simulink model "Kirov_physics"  (R2024b)
settings: Solver=FixedStepDiscrete  StartTime=0.0  StopTime=inf  FixedStep=dt  RelTol=1e-3
undefined symbols (not defined in the file): accel_O, airspeed_bp, alpha_B, alpha_bp, alphaFull, alphaOff, b, battery_capacity_bp, battery_current_bp, battery_initial_capacity_mAh, battery_voltage_table, beta_bp, betaFull, betaOff, brake, brakes, c, channels, CLa, Clb, Clp, CLq, Clr, Cma, Cmq, Cnb, Cnp, Cnr, current_table, DiscIntNeverNeededParam, dt, ELEV_bp, elevator, f, flap, flaps, FLAPS_bp, gear, heightFadeStart, heightOff, hgt_0, Inertia_body, Inertia_load, kInduced, L_aileron, L_throttle, LAILE_bp, lat_0, lon_0, M_aile, M_body, M_elev, M_flap, M_front_gear, M_load, M_main_gear, M_prop, M_rudd, M_spoiler, minWingHeight ... (+36)
libraries: sm_lib x673, simulink x58, nesl_utility x51, simulink_extras x24, uavmavlinklib x12, instrumentlib x4, vrlib x3, aerolibfltsims x3, sharedtransform x3, eeGeneralControl x2, aerolibutil x2, AP_Connector x2
(part 5 of 6)

== system Kirov_physics/Dynamics/Subsystem2 ==
  surface_input(deg) : Inport
  Degrees to Radians : simulink_extras/Transformations/Degrees to Radians
  Discrete Derivative : simulink/Quick Insert/Discrete/Discrete Derivative  gainval=1.0  ICPrevScaledInput=0.0  OutMin=[]  OutMax=[]  OutDataType=fixdt(1, 16)  OutScaling=2^-10  DoSatur=off
  Discrete Derivative1 : simulink/Quick Insert/Discrete/Discrete Derivative  gainval=1.0  ICPrevScaledInput=0.0  OutMin=[]  OutMax=[]  OutDataType=fixdt(1, 16)  OutScaling=2^-10  DoSatur=off
  Simulink-PS Converter : nesl_utility/Simulink-PS Converter  PhysicalDomain=network_engine_domain  SubClassName=ps_input  LeftPortType=input  RightPortType=output  PseudoPeriodic=off  Frequencies=[]  NoiseDistribution=none  NoiseParameters=[]  Unit=rad  AffineConversion=off  FilteringAndDerivatives=provide  SimscapeFilterOrder=1  InputFilterTimeConstant=0.001  UdotUserProvided=2
  surface_output : PMIOPort  Side=Right
  wires:
  Degrees to Radians/1 -> Simulink-PS Converter/1, Discrete Derivative/1
  Discrete Derivative1/1 -> Simulink-PS Converter/3
  Discrete Derivative/1 -> Simulink-PS Converter/2, Discrete Derivative1/1
  surface_input(deg)/1 -> Degrees to Radians/1
  connections:
  Simulink-PS Converter/RConn1 -- surface_output/RConn1

== system Kirov_physics/Dynamics/Subsystem20 ==
  prop_rad : Inport
  Discrete Derivative : simulink/Quick Insert/Discrete/Discrete Derivative  gainval=1.0  ICPrevScaledInput=0.0  OutMin=[]  OutMax=[]  OutDataType=fixdt(1, 16)  OutScaling=2^-10  DoSatur=off
  Discrete Derivative1 : simulink/Quick Insert/Discrete/Discrete Derivative  gainval=1.0  ICPrevScaledInput=0.0  OutMin=[]  OutMax=[]  OutDataType=fixdt(1, 16)  OutScaling=2^-10  DoSatur=off
  Simulink-PS Converter : nesl_utility/Simulink-PS Converter  PhysicalDomain=network_engine_domain  SubClassName=ps_input  LeftPortType=input  RightPortType=output  PseudoPeriodic=off  Frequencies=[]  NoiseDistribution=none  NoiseParameters=[]  Unit=rad  AffineConversion=off  FilteringAndDerivatives=provide  SimscapeFilterOrder=1  InputFilterTimeConstant=0.001  UdotUserProvided=2
  prop_output : PMIOPort  Side=Right
  wires:
  Discrete Derivative/1 -> Discrete Derivative1/1, Simulink-PS Converter/2
  Discrete Derivative1/1 -> Simulink-PS Converter/3
  prop_rad/1 -> Discrete Derivative/1, Simulink-PS Converter/1
  connections:
  Simulink-PS Converter/RConn1 -- prop_output/RConn1

== system Kirov_physics/Dynamics/Subsystem3 ==
  surface_input(deg) : Inport
  Degrees to Radians : simulink_extras/Transformations/Degrees to Radians
  Discrete Derivative : simulink/Quick Insert/Discrete/Discrete Derivative  gainval=1.0  ICPrevScaledInput=0.0  OutMin=[]  OutMax=[]  OutDataType=fixdt(1, 16)  OutScaling=2^-10  DoSatur=off
  Discrete Derivative1 : simulink/Quick Insert/Discrete/Discrete Derivative  gainval=1.0  ICPrevScaledInput=0.0  OutMin=[]  OutMax=[]  OutDataType=fixdt(1, 16)  OutScaling=2^-10  DoSatur=off
  Simulink-PS Converter : nesl_utility/Simulink-PS Converter  PhysicalDomain=network_engine_domain  SubClassName=ps_input  LeftPortType=input  RightPortType=output  PseudoPeriodic=off  Frequencies=[]  NoiseDistribution=none  NoiseParameters=[]  Unit=rad  AffineConversion=off  FilteringAndDerivatives=provide  SimscapeFilterOrder=1  InputFilterTimeConstant=0.001  UdotUserProvided=2
  surface_output : PMIOPort  Side=Right
  wires:
  Degrees to Radians/1 -> Simulink-PS Converter/1, Discrete Derivative/1
  Discrete Derivative1/1 -> Simulink-PS Converter/3
  Discrete Derivative/1 -> Simulink-PS Converter/2, Discrete Derivative1/1
  surface_input(deg)/1 -> Degrees to Radians/1
  connections:
  Simulink-PS Converter/RConn1 -- surface_output/RConn1

== system Kirov_physics/Dynamics/Subsystem4 ==
  surface_input(deg) : Inport
  Degrees to Radians : simulink_extras/Transformations/Degrees to Radians
  Discrete Derivative : simulink/Quick Insert/Discrete/Discrete Derivative  gainval=1.0  ICPrevScaledInput=0.0  OutMin=[]  OutMax=[]  OutDataType=fixdt(1, 16)  OutScaling=2^-10  DoSatur=off
  Discrete Derivative1 : simulink/Quick Insert/Discrete/Discrete Derivative  gainval=1.0  ICPrevScaledInput=0.0  OutMin=[]  OutMax=[]  OutDataType=fixdt(1, 16)  OutScaling=2^-10  DoSatur=off
  Simulink-PS Converter : nesl_utility/Simulink-PS Converter  PhysicalDomain=network_engine_domain  SubClassName=ps_input  LeftPortType=input  RightPortType=output  PseudoPeriodic=off  Frequencies=[]  NoiseDistribution=none  NoiseParameters=[]  Unit=rad  AffineConversion=off  FilteringAndDerivatives=provide  SimscapeFilterOrder=1  InputFilterTimeConstant=0.001  UdotUserProvided=2
  surface_output : PMIOPort  Side=Right
  wires:
  surface_input(deg)/1 -> Degrees to Radians/1
  Discrete Derivative/1 -> Discrete Derivative1/1, Simulink-PS Converter/2
  Discrete Derivative1/1 -> Simulink-PS Converter/3
  Degrees to Radians/1 -> Discrete Derivative/1, Simulink-PS Converter/1
  connections:
  Simulink-PS Converter/RConn1 -- surface_output/RConn1

== system Kirov_physics/Dynamics/Subsystem5 ==
  surface_input(deg) : Inport
  Degrees to Radians : simulink_extras/Transformations/Degrees to Radians
  Discrete Derivative : simulink/Quick Insert/Discrete/Discrete Derivative  gainval=1.0  ICPrevScaledInput=0.0  OutMin=[]  OutMax=[]  OutDataType=fixdt(1, 16)  OutScaling=2^-10  DoSatur=off
  Discrete Derivative1 : simulink/Quick Insert/Discrete/Discrete Derivative  gainval=1.0  ICPrevScaledInput=0.0  OutMin=[]  OutMax=[]  OutDataType=fixdt(1, 16)  OutScaling=2^-10  DoSatur=off
  Simulink-PS Converter : nesl_utility/Simulink-PS Converter  PhysicalDomain=network_engine_domain  SubClassName=ps_input  LeftPortType=input  RightPortType=output  PseudoPeriodic=off  Frequencies=[]  NoiseDistribution=none  NoiseParameters=[]  Unit=rad  AffineConversion=off  FilteringAndDerivatives=provide  SimscapeFilterOrder=1  InputFilterTimeConstant=0.001  UdotUserProvided=2
  surface_output : PMIOPort  Side=Right
  wires:
  surface_input(deg)/1 -> Degrees to Radians/1
  Discrete Derivative/1 -> Discrete Derivative1/1, Simulink-PS Converter/2
  Discrete Derivative1/1 -> Simulink-PS Converter/3
  Degrees to Radians/1 -> Discrete Derivative/1, Simulink-PS Converter/1
  connections:
  Simulink-PS Converter/RConn1 -- surface_output/RConn1

== system Kirov_physics/Dynamics/Subsystem6 ==
  surface_input(deg) : Inport
  Degrees to Radians : simulink_extras/Transformations/Degrees to Radians
  Discrete Derivative : simulink/Quick Insert/Discrete/Discrete Derivative  gainval=1.0  ICPrevScaledInput=0.0  OutMin=[]  OutMax=[]  OutDataType=fixdt(1, 16)  OutScaling=2^-10  DoSatur=off
  Discrete Derivative1 : simulink/Quick Insert/Discrete/Discrete Derivative  gainval=1.0  ICPrevScaledInput=0.0  OutMin=[]  OutMax=[]  OutDataType=fixdt(1, 16)  OutScaling=2^-10  DoSatur=off
  Simulink-PS Converter : nesl_utility/Simulink-PS Converter  PhysicalDomain=network_engine_domain  SubClassName=ps_input  LeftPortType=input  RightPortType=output  PseudoPeriodic=off  Frequencies=[]  NoiseDistribution=none  NoiseParameters=[]  Unit=rad  AffineConversion=off  FilteringAndDerivatives=provide  SimscapeFilterOrder=1  InputFilterTimeConstant=0.001  UdotUserProvided=2
  surface_output : PMIOPort  Side=Right
  wires:
  Degrees to Radians/1 -> Simulink-PS Converter/1, Discrete Derivative/1
  Discrete Derivative1/1 -> Simulink-PS Converter/3
  Discrete Derivative/1 -> Simulink-PS Converter/2, Discrete Derivative1/1
  surface_input(deg)/1 -> Degrees to Radians/1
  connections:
  Simulink-PS Converter/RConn1 -- surface_output/RConn1

== system Kirov_physics/Dynamics/Subsystem7 ==
  force_input(N) : Inport
  Discrete Derivative : simulink/Quick Insert/Discrete/Discrete Derivative  gainval=1.0  ICPrevScaledInput=0.0  OutMin=[]  OutMax=[]  OutDataType=fixdt(1, 16)  OutScaling=2^-10  DoSatur=off
  Discrete Derivative1 : simulink/Quick Insert/Discrete/Discrete Derivative  gainval=1.0  ICPrevScaledInput=0.0  OutMin=[]  OutMax=[]  OutDataType=fixdt(1, 16)  OutScaling=2^-10  DoSatur=off
  Simulink-PS Converter : nesl_utility/Simulink-PS Converter  PhysicalDomain=network_engine_domain  SubClassName=ps_input  LeftPortType=input  RightPortType=output  PseudoPeriodic=off  Frequencies=[]  NoiseDistribution=none  NoiseParameters=[]  Unit=N  AffineConversion=off  FilteringAndDerivatives=provide  SimscapeFilterOrder=1  InputFilterTimeConstant=0.001  UdotUserProvided=2
  force_output : PMIOPort  Side=Right
  wires:
  force_input(N)/1 -> Discrete Derivative/1, Simulink-PS Converter/1
  Discrete Derivative/1 -> Discrete Derivative1/1, Simulink-PS Converter/2
  Discrete Derivative1/1 -> Simulink-PS Converter/3
  connections:
  Simulink-PS Converter/RConn1 -- force_output/RConn1

== system Kirov_physics/Dynamics/Subsystem8 ==
  force_input(N) : Inport
  Discrete Derivative : simulink/Quick Insert/Discrete/Discrete Derivative  gainval=1.0  ICPrevScaledInput=0.0  OutMin=[]  OutMax=[]  OutDataType=fixdt(1, 16)  OutScaling=2^-10  DoSatur=off
  Discrete Derivative1 : simulink/Quick Insert/Discrete/Discrete Derivative  gainval=1.0  ICPrevScaledInput=0.0  OutMin=[]  OutMax=[]  OutDataType=fixdt(1, 16)  OutScaling=2^-10  DoSatur=off
  Simulink-PS Converter : nesl_utility/Simulink-PS Converter  PhysicalDomain=network_engine_domain  SubClassName=ps_input  LeftPortType=input  RightPortType=output  PseudoPeriodic=off  Frequencies=[]  NoiseDistribution=none  NoiseParameters=[]  Unit=N  AffineConversion=off  FilteringAndDerivatives=provide  SimscapeFilterOrder=1  InputFilterTimeConstant=0.001  UdotUserProvided=2
  force_output : PMIOPort  Side=Right
  wires:
  Discrete Derivative1/1 -> Simulink-PS Converter/3
  Discrete Derivative/1 -> Simulink-PS Converter/2, Discrete Derivative1/1
  force_input(N)/1 -> Simulink-PS Converter/1, Discrete Derivative/1
  connections:
  Simulink-PS Converter/RConn1 -- force_output/RConn1

== system Kirov_physics/Dynamics/Subsystem9 ==
  force_input(N) : Inport
  Discrete Derivative : simulink/Quick Insert/Discrete/Discrete Derivative  gainval=1.0  ICPrevScaledInput=0.0  OutMin=[]  OutMax=[]  OutDataType=fixdt(1, 16)  OutScaling=2^-10  DoSatur=off
  Discrete Derivative1 : simulink/Quick Insert/Discrete/Discrete Derivative  gainval=1.0  ICPrevScaledInput=0.0  OutMin=[]  OutMax=[]  OutDataType=fixdt(1, 16)  OutScaling=2^-10  DoSatur=off
  Simulink-PS Converter : nesl_utility/Simulink-PS Converter  PhysicalDomain=network_engine_domain  SubClassName=ps_input  LeftPortType=input  RightPortType=output  PseudoPeriodic=off  Frequencies=[]  NoiseDistribution=none  NoiseParameters=[]  Unit=N  AffineConversion=off  FilteringAndDerivatives=provide  SimscapeFilterOrder=1  InputFilterTimeConstant=0.001  UdotUserProvided=2
  force_output : PMIOPort  Side=Right
  wires:
  force_input(N)/1 -> Discrete Derivative/1, Simulink-PS Converter/1
  Discrete Derivative/1 -> Discrete Derivative1/1, Simulink-PS Converter/2
  Discrete Derivative1/1 -> Simulink-PS Converter/3
  connections:
  Simulink-PS Converter/RConn1 -- force_output/RConn1

== system Kirov_physics/FlightGearView/WGS84 ==
  pos_O_m : Inport
  initial_pos : Inport  Port=2
  Add : Sum
  Data Type Conversion : DataTypeConversion  OutDataTypeStr=double  SaturateOnIntegerOverflow=off  RndMeth=Floor
  Delay : Delay  DelayLength=1
  Delay1 : Delay  DelayLength=1  InitialConditionSource=Input port  InitialCondition=[lat_0;lon_0;hgt_0]
      settings: InputPortMap=u0,p4
  Demux : Demux  Outputs=3
  Divide : Product  Inputs=/*
  Mux : Mux  Inputs=3
  Subtract : Sum  Inputs=+-
  Terminator : Terminator
  WGS84_Derivative : Subsystem
  Zero_Value_Exclusion : Subsystem
  WGS84_Pos : Outport  VectorParamsAs1DForOutWhenUnconnected=off
  wires:
  pos_O_m/1 -> Data Type Conversion/1
  Delay/1 -> Subtract/2
  WGS84_Derivative/1(dx_dlat) -> Mux/1
  Mux/1 -> Zero_Value_Exclusion/1(u)
  Zero_Value_Exclusion/1(y) -> Divide/1
  WGS84_Derivative/3(dz_dh) -> Mux/3
  WGS84_Derivative/2(dy_dlon) -> Mux/2
  Subtract/1 -> Divide/2
  Divide/1 -> Add/1
  Delay1/1 -> Add/2, Demux/1
  Add/1 -> Delay1/1, WGS84_Pos/1
  Demux/1 -> WGS84_Derivative/1(lat_0)
  Demux/3 -> WGS84_Derivative/2(h_0)
  Demux/2 -> Terminator/1
  Data Type Conversion/1 -> Delay/1, Subtract/1
  initial_pos/1 -> Delay1/2

== system Kirov_physics/Referee/Resettable Subsystem ==
  beep : Inport
  Add : Sum
  Constant : Constant  OutDataTypeStr=uint64
  Constant1 : Constant  Value=600
  Delay One Step : Delay  DelayLength=1  InitialCondition=0  ExternalReset=Rising
      settings: InputPortMap=u0,r5
  Enabled Subsystem : Subsystem  TreatAsAtomicUnit=on
  Less Than : RelationalOperator  Operator=<  OutDataTypeStr=boolean  RndMeth=Simplest  InputSameDT=off
  wires:
  Delay One Step/1 -> Add/2
  Constant/1 -> Add/1
  Add/1 -> Less Than/1, Delay One Step/1
  Constant1/1 -> Less Than/2
  Less Than/1 -> Enabled Subsystem/Enable
  beep/1 -> Delay One Step/2

== system Kirov_physics/SendState/Ardupilot ==
  State : Inport
  AP send : AP_Connector/AP send  SystemSampleTime=-1  VariantActivationTime=update diagram  AllowFlexibleInterface=on  Latency=0  AutoFrameSizeCalculation=off
      settings: SourceProductName=AP Connector
  Add Constant : Bias  Bias=[0;0;-9.80665]  SaturateOnIntegerOverflow=off
  Bus Selector1 : BusSelector  OutputSignals=omega_B,q,accel_O,velocity_O,position_O
  Degrees to Radians : simulink_extras/Transformations/Degrees to Radians
  Quaternion Rotation : aerolibutil/Quaternion Rotation
  Quaternions to Rotation Angles : sharedtransform/Quaternions to Rotation Angles  rotationOrder=ZYX  aMode=aMode
  Selector : Selector  InputPortWidth=3  IndexOptions=Index vector (dialog)  Indices=[3 2 1]  OutputSizes=1
  wires:
  Quaternion Rotation/1 -> AP send/3  "accel_B"
  Selector/1 -> AP send/2  "phi_theta_psi"
  Degrees to Radians/1 -> AP send/1  "omega_B"
  State/1 -> Bus Selector1/1
  Bus Selector1/1 -> Degrees to Radians/1  "<omega_B>"
  Bus Selector1/2 -> Quaternion Rotation/1, Quaternions to Rotation Angles/1  "<q>"
  Quaternions to Rotation Angles/1 -> Selector/1
  Bus Selector1/4 -> AP send/4  "<velocity_O>"
  Bus Selector1/5 -> AP send/5  "<position_O>"
  Bus Selector1/3 -> Add Constant/1  "<accel_O>"
  Add Constant/1 -> Quaternion Rotation/2

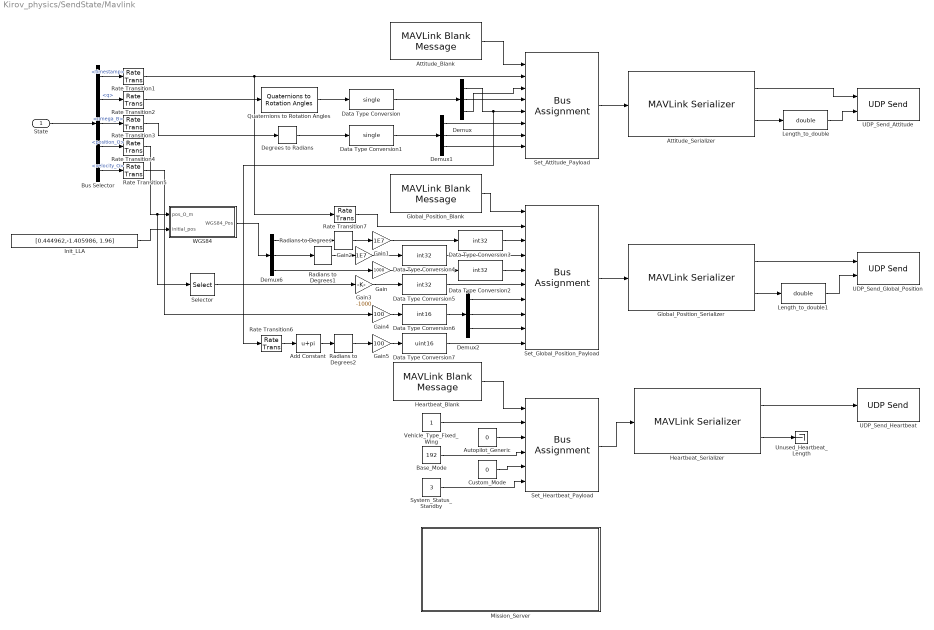
== system Kirov_physics/SendState/Mavlink ==
  State : Inport
  Add Constant : Bias  Bias=pi  SaturateOnIntegerOverflow=off
  Attitude_Blank : uavmavlinklib/MAVLink Blank Message  dialectSource=Select from standard MAVLink dialects  dialect=common.xml  dialectCustom=common.xml  version=2  messageType=ATTITUDE  SystemID=1  ComponentID=1  SampleTime=0.05
  Attitude_Serializer : uavmavlinklib/MAVLink Serializer  dialectSource=Select from standard MAVLink dialects  dialect=common.xml  dialectCustom=common.xml  version=2  messageType=ATTITUDE
  Autopilot_Generic : Constant  Value=0  OutDataTypeStr=uint8
  Base_Mode : Constant  Value=192  OutDataTypeStr=uint8
  Bus Selector : BusSelector  OutputSignals=timestamp,q,omega_B,position_O,velocity_O
  Custom_Mode : Constant  Value=0  OutDataTypeStr=uint32
  Data Type Conversion : DataTypeConversion  OutDataTypeStr=single  SaturateOnIntegerOverflow=off  RndMeth=Floor
  Data Type Conversion1 : DataTypeConversion  OutDataTypeStr=single  SaturateOnIntegerOverflow=off  RndMeth=Floor
  Data Type Conversion{2..5} (4 alike) : DataTypeConversion  OutDataTypeStr=int32  SaturateOnIntegerOverflow=off  RndMeth=Floor
  Data Type Conversion6 : DataTypeConversion  OutDataTypeStr=int16  SaturateOnIntegerOverflow=off  RndMeth=Floor
  Data Type Conversion7 : DataTypeConversion  OutDataTypeStr=uint16  SaturateOnIntegerOverflow=off  RndMeth=Floor
  Degrees to Radians : simulink_extras/Transformations/Degrees to Radians
  Demux{,1..2,6} (4 alike) : Demux  Outputs=3
  Gain : Gain  Gain=1000
  Gain1 : Gain  Gain=1E7
  Gain2 : Gain  Gain=1E7
  Gain3 : Gain  Gain=-1000
  Gain4 : Gain  Gain=100
  Gain5 : Gain  Gain=100
  Global_Position_Blank : uavmavlinklib/MAVLink Blank Message  dialectSource=Select from standard MAVLink dialects  dialect=common.xml  dialectCustom=common.xml  version=2  messageType=GLOBAL_POSITION_INT  SystemID=1  ComponentID=1  SampleTime=0.1
  Global_Position_Serializer : uavmavlinklib/MAVLink Serializer  dialectSource=Select from standard MAVLink dialects  dialect=common.xml  dialectCustom=common.xml  version=2  messageType=GLOBAL_POSITION_INT
  Heartbeat_Blank : uavmavlinklib/MAVLink Blank Message  dialectSource=Select from standard MAVLink dialects  dialect=common.xml  dialectCustom=common.xml  version=2  messageType=HEARTBEAT  SystemID=1  ComponentID=1  SampleTime=1
  Heartbeat_Serializer : uavmavlinklib/MAVLink Serializer  dialectSource=Select from standard MAVLink dialects  dialect=common.xml  dialectCustom=common.xml  version=2  messageType=HEARTBEAT
  Init_LLA : Constant  Value=[0.444962,-1.405986, 1.96]  OutDataTypeStr=double
  Length_to_double : DataTypeConversion  OutDataTypeStr=double  SaturateOnIntegerOverflow=off  RndMeth=Floor
  Length_to_double1 : DataTypeConversion  OutDataTypeStr=double  SaturateOnIntegerOverflow=off  RndMeth=Floor
  Mission_Server : Subsystem
  Quaternions to Rotation Angles : sharedtransform/Quaternions to Rotation Angles  rotationOrder=ZYX  aMode=aMode
  Radians to Degrees : simulink_extras/Transformations/Radians to Degrees
  Radians to Degrees1 : simulink_extras/Transformations/Radians to Degrees
  Radians to Degrees2 : simulink_extras/Transformations/Radians to Degrees
  Rate Transition{1..7} (7 alike) : RateTransition  Integrity=off
  Selector : Selector  InputPortWidth=3  IndexOptions=Index vector (dialog)  Indices=[3]  OutputSizes=1
  Set_Attitude_Payload : BusAssignment  AssignedSignals=Payload.time_boot_ms,Payload.roll,Payload.pitch,Payload.yaw,Payload.rollspeed,Payload.pitchspeed,Payload.yawspeed
  Set_Global_Position_Payload : BusAssignment  AssignedSignals=Payload.time_boot_ms,Payload.lat,Payload.lon,Payload.alt,Payload.relative_alt,Payload.vx,Payload.vy,Payload.vz,Payload.hdg
  Set_Heartbeat_Payload : BusAssignment  AssignedSignals=Payload.type,Payload.autopilot,Payload.base_mode,Payload.custom_mode,Payload.system_status
  System_Status_Standby : Constant  Value=3  OutDataTypeStr=uint8
  UDP_Send_Attitude : dspnetwork/UDP Send  remoteURL='127.0.0.1'  remotePort=14550  localURL='0.0.0.0'  localPortSource=Specify via dialog  localPort=14561  sendBufferSize=8192  sampletime=-1  blockPlatform=[]  separateLengthPort=1
  UDP_Send_Global_Position : dspnetwork/UDP Send  remoteURL='127.0.0.1'  remotePort=14550  localURL='0.0.0.0'  localPortSource=Specify via dialog  localPort=14562  sendBufferSize=8192  sampletime=-1  blockPlatform=[]  separateLengthPort=1
  UDP_Send_Heartbeat : instrumentlib/UDP Send  Host=127.0.0.1  Port=14550  LocalAddress=0.0.0.0  LocalPort=14560  EnablePortSharing=on  OutputDatagramPacketSize=280  ByteOrder=big-endian  EnableBlockingMode=off  SimulateUsing=Interpreted execution
  Unused_Heartbeat_Length : Terminator
  Vehicle_Type_Fixed_Wing : Constant  OutDataTypeStr=uint8
  WGS84 : Subsystem
  wires:
  Set_Attitude_Payload/1 -> Attitude_Serializer/1
  Attitude_Serializer/1 -> UDP_Send_Attitude/1
  Attitude_Serializer/2 -> Length_to_double/1
  Length_to_double/1 -> UDP_Send_Attitude/2
  Attitude_Blank/1 -> Set_Attitude_Payload/1
  Data Type Conversion7/1 -> Set_Global_Position_Payload/10
  Set_Global_Position_Payload/1 -> Global_Position_Serializer/1
  Selector/1 -> Gain3/1
  Global_Position_Blank/1 -> Set_Global_Position_Payload/1
  Global_Position_Serializer/1 -> UDP_Send_Global_Position/1
  Global_Position_Serializer/2 -> Length_to_double1/1
  Length_to_double1/1 -> UDP_Send_Global_Position/2
  Autopilot_Generic/1 -> Set_Heartbeat_Payload/3
  Base_Mode/1 -> Set_Heartbeat_Payload/4
  Vehicle_Type_Fixed_Wing/1 -> Set_Heartbeat_Payload/2
  System_Status_Standby/1 -> Set_Heartbeat_Payload/6
  Heartbeat_Blank/1 -> Set_Heartbeat_Payload/1
  Custom_Mode/1 -> Set_Heartbeat_Payload/5
  State/1 -> Bus Selector/1
  Bus Selector/1 -> Rate Transition1/1  "<timestamp>"
  Bus Selector/4 -> Rate Transition4/1  "<position_O>"
  Bus Selector/5 -> Rate Transition5/1  "<velocity_O>"
  Bus Selector/2 -> Rate Transition2/1  "<q>"
  Bus Selector/3 -> Rate Transition3/1  "<omega_B>"
  Quaternions to Rotation Angles/1 -> Data Type Conversion/1
  Demux/1 -> Rate Transition6/1, Set_Attitude_Payload/5
  Demux/2 -> Set_Attitude_Payload/4
  Demux/3 -> Set_Attitude_Payload/3
  Data Type Conversion/1 -> Demux/1
  Degrees to Radians/1 -> Data Type Conversion1/1
  Data Type Conversion1/1 -> Demux1/1
  Demux1/1 -> Set_Attitude_Payload/6
  Demux1/2 -> Set_Attitude_Payload/7
  Demux1/3 -> Set_Attitude_Payload/8
  Demux6/3 -> Gain/1
  Demux6/1 -> Radians to Degrees/1
  WGS84/1(WGS84_Pos) -> Demux6/1
  Init_LLA/1 -> WGS84/2(initial_pos)
  Gain/1 -> Data Type Conversion2/1
  Data Type Conversion2/1 -> Set_Global_Position_Payload/5
  Radians to Degrees/1 -> Gain1/1
  Gain1/1 -> Data Type Conversion3/1
  Data Type Conversion3/1 -> Set_Global_Position_Payload/3
  Gain2/1 -> Data Type Conversion4/1
  Radians to Degrees1/1 -> Gain2/1
  Demux6/2 -> Radians to Degrees1/1
  Data Type Conversion4/1 -> Set_Global_Position_Payload/4
  Gain3/1 -> Data Type Conversion5/1
  Data Type Conversion5/1 -> Set_Global_Position_Payload/6
  Gain4/1 -> Data Type Conversion6/1
  Data Type Conversion6/1 -> Demux2/1
  Demux2/1 -> Set_Global_Position_Payload/7
  Demux2/2 -> Set_Global_Position_Payload/8
  Demux2/3 -> Set_Global_Position_Payload/9
  Gain5/1 -> Data Type Conversion7/1
  Radians to Degrees2/1 -> Gain5/1
  Rate Transition1/1 -> Set_Attitude_Payload/2, Rate Transition7/1
  Rate Transition2/1 -> Quaternions to Rotation Angles/1
  Rate Transition3/1 -> Degrees to Radians/1
  Rate Transition4/1 -> Selector/1, WGS84/1(pos_O_m)
  Rate Transition5/1 -> Gain4/1
  Rate Transition6/1 -> Add Constant/1
  Rate Transition7/1 -> Set_Global_Position_Payload/2
  Add Constant/1 -> Radians to Degrees2/1
  Heartbeat_Serializer/2 -> Unused_Heartbeat_Length/1
  Heartbeat_Serializer/1 -> UDP_Send_Heartbeat/1
  Set_Heartbeat_Payload/1 -> Heartbeat_Serializer/1

== system Kirov_physics/wind_NED/timestamp ==
  Constant : Constant  Value=sample_time
  Data Type Conversion : DataTypeConversion  OutDataTypeStr=uint32  SaturateOnIntegerOverflow=off  RndMeth=Floor
  Discrete-Time Integrator : DiscreteIntegrator  IntegratorMethod=Accumulation: Forward Euler  SampleTime=-1  ICPrevOutput=DiscIntNeverNeededParam  ICPrevScaledInput=DiscIntNeverNeededParam
  timestamp_ms : Outport  VectorParamsAs1DForOutWhenUnconnected=off
  wires:
  Discrete-Time Integrator/1 -> Data Type Conversion/1
  Constant/1 -> Discrete-Time Integrator/1
  Data Type Conversion/1 -> timestamp_ms/1

== system Kirov_physics/Actuator/Subsystem1/dynamic_rate_saturation ==
  control_in : Inport
  rate : Inport  Port=2
  Delay : Delay  DelayLength=1  InitialConditionSource=Input port
      settings: InputPortMap=u0,p4
  Gain : Gain  Gain=dt
  Gain3 : Gain  Gain=-1
  Saturation Dynamic : simulink/Discontinuities/Saturation Dynamic  OutMin=[]  OutMax=[]  OutDataTypeStr=Inherit: Same as second input  OutDataType=fixdt(1, 16)  OutScaling=2^-10  DoSatur=off
  Sum : Sum  Inputs=|++
  subtract1 : Sum  Inputs=+-
  control_out : Outport  VectorParamsAs1DForOutWhenUnconnected=off
  wires:
  Sum/1 -> Delay/1
  Delay/1 -> control_out/1, subtract1/2, Sum/2
  control_in/1 -> Delay/2, subtract1/1
  subtract1/1 -> Saturation Dynamic/2
  Saturation Dynamic/1 -> Sum/1
  rate/1 -> Gain/1
  Gain3/1 -> Saturation Dynamic/3
  Gain/1 -> Saturation Dynamic/1, Gain3/1

== system Kirov_physics/Actuator/Subsystem2/dynamic_rate_saturation ==
  control_in : Inport
  rate : Inport  Port=2
  Delay : Delay  DelayLength=1  InitialConditionSource=Input port
      settings: InputPortMap=u0,p4
  Gain : Gain  Gain=dt
  Gain3 : Gain  Gain=-1
  Saturation Dynamic : simulink/Discontinuities/Saturation Dynamic  OutMin=[]  OutMax=[]  OutDataTypeStr=Inherit: Same as second input  OutDataType=fixdt(1, 16)  OutScaling=2^-10  DoSatur=off
  Sum : Sum  Inputs=|++
  subtract1 : Sum  Inputs=+-
  control_out : Outport  VectorParamsAs1DForOutWhenUnconnected=off
  wires:
  Gain/1 -> Gain3/1, Saturation Dynamic/1
  Gain3/1 -> Saturation Dynamic/3
  rate/1 -> Gain/1
  Saturation Dynamic/1 -> Sum/1
  subtract1/1 -> Saturation Dynamic/2
  control_in/1 -> subtract1/1, Delay/2
  Delay/1 -> Sum/2, subtract1/2, control_out/1
  Sum/1 -> Delay/1

== system Kirov_physics/Actuator/Subsystem3/dynamic_rate_saturation ==
  control_in : Inport
  rate : Inport  Port=2
  Delay : Delay  DelayLength=1  InitialConditionSource=Input port
      settings: InputPortMap=u0,p4
  Gain : Gain  Gain=dt
  Gain3 : Gain  Gain=-1
  Saturation Dynamic : simulink/Discontinuities/Saturation Dynamic  OutMin=[]  OutMax=[]  OutDataTypeStr=Inherit: Same as second input  OutDataType=fixdt(1, 16)  OutScaling=2^-10  DoSatur=off
  Sum : Sum  Inputs=|++
  subtract1 : Sum  Inputs=+-
  control_out : Outport  VectorParamsAs1DForOutWhenUnconnected=off
  wires:
  Sum/1 -> Delay/1
  Delay/1 -> control_out/1, subtract1/2, Sum/2
  control_in/1 -> Delay/2, subtract1/1
  subtract1/1 -> Saturation Dynamic/2
  Saturation Dynamic/1 -> Sum/1
  rate/1 -> Gain/1
  Gain3/1 -> Saturation Dynamic/3
  Gain/1 -> Saturation Dynamic/1, Gain3/1

== system Kirov_physics/Actuator/Subsystem4/dynamic_rate_saturation ==
  control_in : Inport
  rate : Inport  Port=2
  Delay : Delay  DelayLength=1  InitialConditionSource=Input port
      settings: InputPortMap=u0,p4
  Gain : Gain  Gain=dt
  Gain3 : Gain  Gain=-1
  Saturation Dynamic : simulink/Discontinuities/Saturation Dynamic  OutMin=[]  OutMax=[]  OutDataTypeStr=Inherit: Same as second input  OutDataType=fixdt(1, 16)  OutScaling=2^-10  DoSatur=off
  Sum : Sum  Inputs=|++
  subtract1 : Sum  Inputs=+-
  control_out : Outport  VectorParamsAs1DForOutWhenUnconnected=off
  wires:
  Gain/1 -> Gain3/1, Saturation Dynamic/1
  Gain3/1 -> Saturation Dynamic/3
  rate/1 -> Gain/1
  Saturation Dynamic/1 -> Sum/1
  subtract1/1 -> Saturation Dynamic/2
  control_in/1 -> subtract1/1, Delay/2
  Delay/1 -> Sum/2, subtract1/2, control_out/1
  Sum/1 -> Delay/1

== system Kirov_physics/Actuator/Subsystem5/dynamic_rate_saturation ==
  control_in : Inport
  rate : Inport  Port=2
  Delay : Delay  DelayLength=1  InitialConditionSource=Input port
      settings: InputPortMap=u0,p4
  Gain : Gain  Gain=dt
  Gain3 : Gain  Gain=-1
  Saturation Dynamic : simulink/Discontinuities/Saturation Dynamic  OutMin=[]  OutMax=[]  OutDataTypeStr=Inherit: Same as second input  OutDataType=fixdt(1, 16)  OutScaling=2^-10  DoSatur=off
  Sum : Sum  Inputs=|++
  subtract1 : Sum  Inputs=+-
  control_out : Outport  VectorParamsAs1DForOutWhenUnconnected=off
  wires:
  Sum/1 -> Delay/1
  Delay/1 -> control_out/1, subtract1/2, Sum/2
  control_in/1 -> Delay/2, subtract1/1
  subtract1/1 -> Saturation Dynamic/2
  Saturation Dynamic/1 -> Sum/1
  rate/1 -> Gain/1
  Gain3/1 -> Saturation Dynamic/3
  Gain/1 -> Saturation Dynamic/1, Gain3/1

== system Kirov_physics/Actuator/Subsystem6/dynamic_rate_saturation ==
  control_in : Inport
  rate : Inport  Port=2
  Delay : Delay  DelayLength=1  InitialConditionSource=Input port
      settings: InputPortMap=u0,p4
  Gain : Gain  Gain=dt
  Gain3 : Gain  Gain=-1
  Saturation Dynamic : simulink/Discontinuities/Saturation Dynamic  OutMin=[]  OutMax=[]  OutDataTypeStr=Inherit: Same as second input  OutDataType=fixdt(1, 16)  OutScaling=2^-10  DoSatur=off
  Sum : Sum  Inputs=|++
  subtract1 : Sum  Inputs=+-
  control_out : Outport  VectorParamsAs1DForOutWhenUnconnected=off
  wires:
  Gain/1 -> Gain3/1, Saturation Dynamic/1
  Gain3/1 -> Saturation Dynamic/3
  rate/1 -> Gain/1
  Saturation Dynamic/1 -> Sum/1
  subtract1/1 -> Saturation Dynamic/2
  control_in/1 -> subtract1/1, Delay/2
  Delay/1 -> Sum/2, subtract1/2, control_out/1
  Sum/1 -> Delay/1

== system Kirov_physics/Actuator/Subsystem7/dynamic_rate_saturation ==
  control_in : Inport
  rate : Inport  Port=2
  Delay : Delay  DelayLength=1  InitialConditionSource=Input port
      settings: InputPortMap=u0,p4
  Gain : Gain  Gain=dt
  Gain3 : Gain  Gain=-1
  Saturation Dynamic : simulink/Discontinuities/Saturation Dynamic  OutMin=[]  OutMax=[]  OutDataTypeStr=Inherit: Same as second input  OutDataType=fixdt(1, 16)  OutScaling=2^-10  DoSatur=off
  Sum : Sum  Inputs=|++
  subtract1 : Sum  Inputs=+-
  control_out : Outport  VectorParamsAs1DForOutWhenUnconnected=off
  wires:
  Sum/1 -> Delay/1
  Delay/1 -> control_out/1, subtract1/2, Sum/2
  control_in/1 -> Delay/2, subtract1/1
  subtract1/1 -> Saturation Dynamic/2
  Saturation Dynamic/1 -> Sum/1
  rate/1 -> Gain/1
  Gain3/1 -> Saturation Dynamic/3
  Gain/1 -> Saturation Dynamic/1, Gain3/1

== system Kirov_physics/Actuator/Subsystem8/dynamic_rate_saturation ==
  control_in : Inport
  rate : Inport  Port=2
  Delay : Delay  DelayLength=1  InitialConditionSource=Input port
      settings: InputPortMap=u0,p4
  Gain : Gain  Gain=dt
  Gain3 : Gain  Gain=-1
  Saturation Dynamic : simulink/Discontinuities/Saturation Dynamic  OutMin=[]  OutMax=[]  OutDataTypeStr=Inherit: Same as second input  OutDataType=fixdt(1, 16)  OutScaling=2^-10  DoSatur=off
  Sum : Sum  Inputs=|++
  subtract1 : Sum  Inputs=+-
  control_out : Outport  VectorParamsAs1DForOutWhenUnconnected=off
  wires:
  Gain/1 -> Gain3/1, Saturation Dynamic/1
  Gain3/1 -> Saturation Dynamic/3
  rate/1 -> Gain/1
  Saturation Dynamic/1 -> Sum/1
  subtract1/1 -> Saturation Dynamic/2
  control_in/1 -> subtract1/1, Delay/2
  Delay/1 -> Sum/2, subtract1/2, control_out/1
  Sum/1 -> Delay/1

== system Kirov_physics/Aerodynamics/GroundEffectCorrection/ApplyGroundEffect ==
  fmBaseBody : Inport
  aeroAnglesDeg : Inport  Port=2
  positionO : Inport  Port=3
  GE_Enable : Inport  Port=4
  refQ : Inport  Port=5
  ApplyInfluence : Subsystem
  BodyToWind : Subsystem
  ComputeWeights : Subsystem
  RotateBackBlend : Subsystem
  fmBaseBodyGE : Outport
  wires:
  BodyToWind/3(CD) -> ApplyInfluence/3(CD)
  aeroAnglesDeg/1 -> ComputeWeights/1(aeroAnglesDeg), BodyToWind/2(aeroAnglesDeg)
  BodyToWind/1(fwind) -> ApplyInfluence/1(fwind)
  BodyToWind/2(CL) -> ApplyInfluence/2(CL), RotateBackBlend/6(CL)
  fmBaseBody/1 -> BodyToWind/1(fmBaseBody), RotateBackBlend/3(fmBaseBody)
  BodyToWind/5(aspectRatio) -> ApplyInfluence/5(aspectRatio)
  positionO/1 -> ComputeWeights/2(positionO)
  BodyToWind/4(qRefS) -> ApplyInfluence/4(qRefS)
  BodyToWind/6(R) -> RotateBackBlend/2(R)
  RotateBackBlend/1(fmBaseBodyGE) -> fmBaseBodyGE/1
  ComputeWeights/2(heightRatio) -> ApplyInfluence/7(heightRatio)
  ComputeWeights/1(correctionWeight) -> RotateBackBlend/5(correctionWeight), ApplyInfluence/6(correctionWeight)
  ApplyInfluence/1(fwindGE) -> RotateBackBlend/1(fwindGE)
  GE_Enable/1 -> RotateBackBlend/4(GE_Enable)
  refQ/1 -> BodyToWind/3(refQ)

== system Kirov_physics/Aerodynamics/propulsion/L_propeller ==
  throttle : Inport
  voltage : Inport  Port=2
  Vx : Inport  Port=3
  Current : Lookup_n-D  NumberOfTableDimensions=3  BreakpointsForDimension1=throttle_bp  BreakpointsForDimension2=voltage_bp  BreakpointsForDimension3=airspeed_bp  BeginIndexSearchUsingPreviousIndexResult=on  Table=current_table  InterpMethod=Linear Lagrange  DiagnosticForOutOfRangeInput=Warning  InternalRulePriority=Speed  RndMeth=Simplest
      settings: InputPortMap=u0,u1,u2
  RPM : Lookup_n-D  NumberOfTableDimensions=3  BreakpointsForDimension1=throttle_bp  BreakpointsForDimension2=voltage_bp  BreakpointsForDimension3=airspeed_bp  BeginIndexSearchUsingPreviousIndexResult=on  Table=rpm_table  InterpMethod=Linear Lagrange  DiagnosticForOutOfRangeInput=Warning  InternalRulePriority=Speed  RndMeth=Simplest
      settings: InputPortMap=u0,u1,u2
  Thrust : Lookup_n-D  NumberOfTableDimensions=3  BreakpointsForDimension1=throttle_bp  BreakpointsForDimension2=voltage_bp  BreakpointsForDimension3=airspeed_bp  BeginIndexSearchUsingPreviousIndexResult=on  Table=thrust_table  InterpMethod=Linear Lagrange  DiagnosticForOutOfRangeInput=Warning  InternalRulePriority=Speed  RndMeth=Simplest
      settings: InputPortMap=u0,u1,u2
  Torque : Lookup_n-D  NumberOfTableDimensions=3  BreakpointsForDimension1=throttle_bp  BreakpointsForDimension2=voltage_bp  BreakpointsForDimension3=airspeed_bp  BeginIndexSearchUsingPreviousIndexResult=on  Table=torque_table  InterpMethod=Linear Lagrange  DiagnosticForOutOfRangeInput=Warning  InternalRulePriority=Speed  RndMeth=Simplest
      settings: InputPortMap=u0,u1,u2
  thrust : Outport
  torque : Outport  Port=2
  rpm : Outport  Port=3
  current : Outport  Port=4
  wires:
  Vx/1 -> Torque/3, Current/3, RPM/3, Thrust/3
  voltage/1 -> Current/2, RPM/2, Torque/2, Thrust/2
  throttle/1 -> Current/1, RPM/1, Torque/1, Thrust/1
  RPM/1 -> rpm/1
  Torque/1 -> torque/1
  Thrust/1 -> thrust/1
  Current/1 -> current/1

== system Kirov_physics/Aerodynamics/propulsion/R_propeller ==
  throttle : Inport
  voltage : Inport  Port=2
  Vx : Inport  Port=3
  Current : Lookup_n-D  NumberOfTableDimensions=3  BreakpointsForDimension1=throttle_bp  BreakpointsForDimension2=voltage_bp  BreakpointsForDimension3=airspeed_bp  BeginIndexSearchUsingPreviousIndexResult=on  Table=current_table  InterpMethod=Linear Lagrange  DiagnosticForOutOfRangeInput=Warning  InternalRulePriority=Speed  RndMeth=Simplest
      settings: InputPortMap=u0,u1,u2
  RPM : Lookup_n-D  NumberOfTableDimensions=3  BreakpointsForDimension1=throttle_bp  BreakpointsForDimension2=voltage_bp  BreakpointsForDimension3=airspeed_bp  BeginIndexSearchUsingPreviousIndexResult=on  Table=rpm_table  InterpMethod=Linear Lagrange  DiagnosticForOutOfRangeInput=Warning  InternalRulePriority=Speed  RndMeth=Simplest
      settings: InputPortMap=u0,u1,u2
  Thrust : Lookup_n-D  NumberOfTableDimensions=3  BreakpointsForDimension1=throttle_bp  BreakpointsForDimension2=voltage_bp  BreakpointsForDimension3=airspeed_bp  BeginIndexSearchUsingPreviousIndexResult=on  Table=thrust_table  InterpMethod=Linear Lagrange  DiagnosticForOutOfRangeInput=Warning  InternalRulePriority=Speed  RndMeth=Simplest
      settings: InputPortMap=u0,u1,u2
  Torque : Lookup_n-D  NumberOfTableDimensions=3  BreakpointsForDimension1=throttle_bp  BreakpointsForDimension2=voltage_bp  BreakpointsForDimension3=airspeed_bp  BeginIndexSearchUsingPreviousIndexResult=on  Table=torque_table  InterpMethod=Linear Lagrange  DiagnosticForOutOfRangeInput=Warning  InternalRulePriority=Speed  RndMeth=Simplest
      settings: InputPortMap=u0,u1,u2
  thrust : Outport
  torque : Outport  Port=2
  rpm : Outport  Port=3
  current : Outport  Port=4
  wires:
  Current/1 -> current/1
  Thrust/1 -> thrust/1
  Torque/1 -> torque/1
  RPM/1 -> rpm/1
  throttle/1 -> Thrust/1, Torque/1, RPM/1, Current/1
  voltage/1 -> Thrust/2, Torque/2, RPM/2, Current/2
  Vx/1 -> Thrust/3, RPM/3, Current/3, Torque/3

== system Kirov_physics/Control_Input/Ardupilot/timestamp1 ==
  Constant : Constant  Value=sample_time
  Data Type Conversion : DataTypeConversion  OutDataTypeStr=uint32  SaturateOnIntegerOverflow=off  RndMeth=Floor
  Discrete-Time Integrator : DiscreteIntegrator  IntegratorMethod=Accumulation: Forward Euler  SampleTime=-1  ICPrevOutput=DiscIntNeverNeededParam  ICPrevScaledInput=DiscIntNeverNeededParam
  timestamp_ms : Outport  VectorParamsAs1DForOutWhenUnconnected=off
  wires:
  Data Type Conversion/1 -> timestamp_ms/1
  Constant/1 -> Discrete-Time Integrator/1
  Discrete-Time Integrator/1 -> Data Type Conversion/1

== system Kirov_physics/Control_Input/Joystick/timestamp1 ==
  Constant : Constant  Value=sample_time
  Data Type Conversion : DataTypeConversion  OutDataTypeStr=uint32  SaturateOnIntegerOverflow=off  RndMeth=Floor
  Discrete-Time Integrator : DiscreteIntegrator  IntegratorMethod=Accumulation: Forward Euler  SampleTime=-1  ICPrevOutput=DiscIntNeverNeededParam  ICPrevScaledInput=DiscIntNeverNeededParam
  timestamp_ms : Outport  VectorParamsAs1DForOutWhenUnconnected=off
  wires:
  Data Type Conversion/1 -> timestamp_ms/1
  Constant/1 -> Discrete-Time Integrator/1
  Discrete-Time Integrator/1 -> Data Type Conversion/1

== system Kirov_physics/Dynamics/Subsystem13/Subsystem13 ==
  surface_input : Inport
  Discrete Derivative : simulink/Quick Insert/Discrete/Discrete Derivative  gainval=1.0  ICPrevScaledInput=0.0  OutMin=[]  OutMax=[]  OutDataType=fixdt(1, 16)  OutScaling=2^-10  DoSatur=off
  Discrete Derivative1 : simulink/Quick Insert/Discrete/Discrete Derivative  gainval=1.0  ICPrevScaledInput=0.0  OutMin=[]  OutMax=[]  OutDataType=fixdt(1, 16)  OutScaling=2^-10  DoSatur=off
  Simulink-PS Converter : nesl_utility/Simulink-PS Converter  PhysicalDomain=network_engine_domain  SubClassName=ps_input  LeftPortType=input  RightPortType=output  PseudoPeriodic=off  Frequencies=[]  NoiseDistribution=none  NoiseParameters=[]  Unit=m  AffineConversion=off  FilteringAndDerivatives=provide  SimscapeFilterOrder=1  InputFilterTimeConstant=0.001  UdotUserProvided=2
  surface_output : PMIOPort  Side=Right
  wires:
  surface_input/1 -> Simulink-PS Converter/1, Discrete Derivative/1
  Discrete Derivative/1 -> Discrete Derivative1/1, Simulink-PS Converter/2
  Discrete Derivative1/1 -> Simulink-PS Converter/3
  connections:
  Simulink-PS Converter/RConn1 -- surface_output/RConn1

== system Kirov_physics/Dynamics/Subsystem13/Subsystem14 ==
  surface_input : Inport
  Discrete Derivative : simulink/Quick Insert/Discrete/Discrete Derivative  gainval=1.0  ICPrevScaledInput=0.0  OutMin=[]  OutMax=[]  OutDataType=fixdt(1, 16)  OutScaling=2^-10  DoSatur=off
  Discrete Derivative1 : simulink/Quick Insert/Discrete/Discrete Derivative  gainval=1.0  ICPrevScaledInput=0.0  OutMin=[]  OutMax=[]  OutDataType=fixdt(1, 16)  OutScaling=2^-10  DoSatur=off
  Simulink-PS Converter : nesl_utility/Simulink-PS Converter  PhysicalDomain=network_engine_domain  SubClassName=ps_input  LeftPortType=input  RightPortType=output  PseudoPeriodic=off  Frequencies=[]  NoiseDistribution=none  NoiseParameters=[]  Unit=m  AffineConversion=off  FilteringAndDerivatives=provide  SimscapeFilterOrder=1  InputFilterTimeConstant=0.001  UdotUserProvided=2
  surface_output : PMIOPort  Side=Right
  wires:
  Discrete Derivative1/1 -> Simulink-PS Converter/3
  Discrete Derivative/1 -> Simulink-PS Converter/2, Discrete Derivative1/1
  surface_input/1 -> Discrete Derivative/1, Simulink-PS Converter/1
  connections:
  Simulink-PS Converter/RConn1 -- surface_output/RConn1

== system Kirov_physics/Dynamics/Subsystem13/Subsystem15 ==
  surface_input : Inport
  Discrete Derivative : simulink/Quick Insert/Discrete/Discrete Derivative  gainval=1.0  ICPrevScaledInput=0.0  OutMin=[]  OutMax=[]  OutDataType=fixdt(1, 16)  OutScaling=2^-10  DoSatur=off
  Discrete Derivative1 : simulink/Quick Insert/Discrete/Discrete Derivative  gainval=1.0  ICPrevScaledInput=0.0  OutMin=[]  OutMax=[]  OutDataType=fixdt(1, 16)  OutScaling=2^-10  DoSatur=off
  Simulink-PS Converter : nesl_utility/Simulink-PS Converter  PhysicalDomain=network_engine_domain  SubClassName=ps_input  LeftPortType=input  RightPortType=output  PseudoPeriodic=off  Frequencies=[]  NoiseDistribution=none  NoiseParameters=[]  Unit=rad  AffineConversion=off  FilteringAndDerivatives=provide  SimscapeFilterOrder=1  InputFilterTimeConstant=0.001  UdotUserProvided=2
  surface_output : PMIOPort  Side=Right
  wires:
  surface_input/1 -> Simulink-PS Converter/1, Discrete Derivative/1
  Discrete Derivative/1 -> Discrete Derivative1/1, Simulink-PS Converter/2
  Discrete Derivative1/1 -> Simulink-PS Converter/3
  connections:
  Simulink-PS Converter/RConn1 -- surface_output/RConn1

== system Kirov_physics/Dynamics/Subsystem16/Subsystem13 ==
  surface_input : Inport
  Discrete Derivative : simulink/Quick Insert/Discrete/Discrete Derivative  gainval=1.0  ICPrevScaledInput=0.0  OutMin=[]  OutMax=[]  OutDataType=fixdt(1, 16)  OutScaling=2^-10  DoSatur=off
  Discrete Derivative1 : simulink/Quick Insert/Discrete/Discrete Derivative  gainval=1.0  ICPrevScaledInput=0.0  OutMin=[]  OutMax=[]  OutDataType=fixdt(1, 16)  OutScaling=2^-10  DoSatur=off
  Simulink-PS Converter : nesl_utility/Simulink-PS Converter  PhysicalDomain=network_engine_domain  SubClassName=ps_input  LeftPortType=input  RightPortType=output  PseudoPeriodic=off  Frequencies=[]  NoiseDistribution=none  NoiseParameters=[]  Unit=m  AffineConversion=off  FilteringAndDerivatives=provide  SimscapeFilterOrder=1  InputFilterTimeConstant=0.001  UdotUserProvided=2
  surface_output : PMIOPort  Side=Right
  wires:
  Discrete Derivative1/1 -> Simulink-PS Converter/3
  Discrete Derivative/1 -> Simulink-PS Converter/2, Discrete Derivative1/1
  surface_input/1 -> Discrete Derivative/1, Simulink-PS Converter/1
  connections:
  Simulink-PS Converter/RConn1 -- surface_output/RConn1

== system Kirov_physics/Dynamics/Subsystem16/Subsystem14 ==
  surface_input : Inport
  Discrete Derivative : simulink/Quick Insert/Discrete/Discrete Derivative  gainval=1.0  ICPrevScaledInput=0.0  OutMin=[]  OutMax=[]  OutDataType=fixdt(1, 16)  OutScaling=2^-10  DoSatur=off
  Discrete Derivative1 : simulink/Quick Insert/Discrete/Discrete Derivative  gainval=1.0  ICPrevScaledInput=0.0  OutMin=[]  OutMax=[]  OutDataType=fixdt(1, 16)  OutScaling=2^-10  DoSatur=off
  Simulink-PS Converter : nesl_utility/Simulink-PS Converter  PhysicalDomain=network_engine_domain  SubClassName=ps_input  LeftPortType=input  RightPortType=output  PseudoPeriodic=off  Frequencies=[]  NoiseDistribution=none  NoiseParameters=[]  Unit=m  AffineConversion=off  FilteringAndDerivatives=provide  SimscapeFilterOrder=1  InputFilterTimeConstant=0.001  UdotUserProvided=2
  surface_output : PMIOPort  Side=Right
  wires:
  surface_input/1 -> Simulink-PS Converter/1, Discrete Derivative/1
  Discrete Derivative/1 -> Discrete Derivative1/1, Simulink-PS Converter/2
  Discrete Derivative1/1 -> Simulink-PS Converter/3
  connections:
  Simulink-PS Converter/RConn1 -- surface_output/RConn1

== system Kirov_physics/Dynamics/Subsystem16/Subsystem15 ==
  surface_input : Inport
  Discrete Derivative : simulink/Quick Insert/Discrete/Discrete Derivative  gainval=1.0  ICPrevScaledInput=0.0  OutMin=[]  OutMax=[]  OutDataType=fixdt(1, 16)  OutScaling=2^-10  DoSatur=off
  Discrete Derivative1 : simulink/Quick Insert/Discrete/Discrete Derivative  gainval=1.0  ICPrevScaledInput=0.0  OutMin=[]  OutMax=[]  OutDataType=fixdt(1, 16)  OutScaling=2^-10  DoSatur=off
  Simulink-PS Converter : nesl_utility/Simulink-PS Converter  PhysicalDomain=network_engine_domain  SubClassName=ps_input  LeftPortType=input  RightPortType=output  PseudoPeriodic=off  Frequencies=[]  NoiseDistribution=none  NoiseParameters=[]  Unit=rad  AffineConversion=off  FilteringAndDerivatives=provide  SimscapeFilterOrder=1  InputFilterTimeConstant=0.001  UdotUserProvided=2
  surface_output : PMIOPort  Side=Right
  wires:
  Discrete Derivative1/1 -> Simulink-PS Converter/3
  Discrete Derivative/1 -> Simulink-PS Converter/2, Discrete Derivative1/1
  surface_input/1 -> Discrete Derivative/1, Simulink-PS Converter/1
  connections:
  Simulink-PS Converter/RConn1 -- surface_output/RConn1

== system Kirov_physics/FlightGearView/WGS84/WGS84_Derivative ==
  lat_0 : Inport
  h_0 : Inport  Port=2
  Add : Sum
  Add1 : Sum
  Divide : Product  Inputs=*/
  Product{,1..4} (5 alike) : Product  RndMeth=Zero
  Subtract : Sum  Inputs=+-
  Subtract1 : Sum  Inputs=-+
  Subtract2 : Sum  Inputs=+-
  Trigonometric Function : Trigonometry
  Trigonometric Function1 : Trigonometry  Operator=cos
  Trigonometric Function2 : Trigonometry  Operator=cos
  b : Constant  Value=1/298.257
  c : Constant
  constant : Constant  Value=2
  constant1 : Constant  Value=-1
  constant2 : Constant
  earth_radius : Constant  Value=6378137
  sqrt : Math  Operator=sqrt  SignedPower=on
  u^1 : Math  Operator=square  SignedPower=on
  u^2 : Math  Operator=square  SignedPower=on
  dx_dlat : Outport  VectorParamsAs1DForOutWhenUnconnected=off
  dy_dlon : Outport  Port=2  VectorParamsAs1DForOutWhenUnconnected=off
  dz_dh : Outport  Port=3  InitialOutput=1  VectorParamsAs1DForOutWhenUnconnected=off
  wires:
  constant1/1 -> dz_dh/1
  Product4/1 -> dy_dlon/1
  Add1/1 -> Product4/1
  Trigonometric Function2/1 -> Product4/2
  Product3/1 -> Add/1
  Subtract2/1 -> Product3/1
  Product2/1 -> Subtract2/2
  u^1/1 -> Product2/1
  Trigonometric Function1/1 -> u^1/1
  constant2/1 -> Subtract2/1
  h_0/1 -> Add1/1, Add/2
  Add/1 -> dx_dlat/1
  Divide/1 -> Product3/2, Add1/2
  sqrt/1 -> Divide/2
  Product1/1 -> Product2/2, Product/1
  Subtract1/1 -> Product1/2
  constant/1 -> Subtract1/2
  b/1 -> Subtract1/1, Product1/1
  Product/1 -> Subtract/2
  Subtract/1 -> sqrt/1
  c/1 -> Subtract/1
  u^2/1 -> Product/2
  Trigonometric Function/1 -> u^2/1
  lat_0/1 -> Trigonometric Function2/1, Trigonometric Function/1, Trigonometric Function1/1
  earth_radius/1 -> Divide/1

== system Kirov_physics/FlightGearView/WGS84/Zero_Value_Exclusion ==
  u : Inport
  Abs : Abs  SaturateOnIntegerOverflow=off
  Constant : Constant
  Product : Product  RndMeth=Zero
  Saturation : Saturate  UpperLimit=10e7  LowerLimit=1e-6  LinearizeAsGain=off
  Sign : Signum
  Switch : Switch  Criteria=u2 ~= 0  SaturateOnIntegerOverflow=off  InputSameDT=off
  y : Outport  VectorParamsAs1DForOutWhenUnconnected=off
  wires:
  u/1 -> Sign/1, Abs/1
  Abs/1 -> Saturation/1
  Saturation/1 -> Product/1
  Sign/1 -> Switch/2, Switch/1
  Product/1 -> y/1
  Switch/1 -> Product/2
  Constant/1 -> Switch/3

== system Kirov_physics/Referee/Resettable Subsystem/Enabled Subsystem ==
  Enable : EnablePort
  Audio Device Writer : dspsnks4/Audio Device Writer  Driver=DirectSound  Device=Default  InheritSampleRate=on  SampleRate=44100  BitDepth=16-bit integer  BufferSize=4096  NumBuffers=10  DefaultOutputChannelMapping=on  OutputChannelMapping=1:2  OutputNumUnderrunSamples=off  DriverIdx=1  DeviceWarnFlag=''
  Buffer : Buffer  N=128  OutputFrames=off
  Signal From Workspace : dspsrcs4/Signal From Workspace  X=alarm  Ts=1/8000  nsamps=8  OutputAfterFinalValue=Cyclic repetition  ignoreOrWarnInputAndFrameLengths=off  OutputFrames=off
  wires:
  Signal From Workspace/1 -> Buffer/1
  Buffer/1 -> Audio Device Writer/1

== system Kirov_physics/SendState/Mavlink/Mission_Server ==
  Decode_Request_Item : uavmavlinklib/MAVLink Deserializer  dialectSource=Select from standard MAVLink dialects  dialect=common.xml  dialectCustom=common.xml  version=2  messageType=MISSION_REQUEST_INT  inputDataLength=off  SystemIDFilter=off  systemID=1  ComponentIDFilter=off  componentID=1  queueMsg=off  queueMsgSize=50  dropNum=off
  Decode_Request_List : uavmavlinklib/MAVLink Deserializer  dialectSource=Select from standard MAVLink dialects  dialect=common.xml  dialectCustom=common.xml  version=2  messageType=MISSION_REQUEST_LIST  inputDataLength=off  SystemIDFilter=off  systemID=1  ComponentIDFilter=off  componentID=1  queueMsg=off  queueMsgSize=50  dropNum=off
  Select_Request_Seq : BusSelector  OutputSignals=Payload.seq
  Send_Mission_Count : Subsystem  TreatAsAtomicUnit=on
  Send_Mission_Item : Subsystem  TreatAsAtomicUnit=on
  UDP_Receive_QGC : instrumentlib/UDP Receive  LocalAddress=0.0.0.0  LocalPort=14560  EnablePortSharing=on  Host=127.0.0.1  Port=14550  GetLatestData=off  DataSize=[1,280]  DataType=uint8  ASCIIFormatting=%f,  Terminator=LF  CustomTerminator=10  ByteOrder=big-endian  EnableBlockingMode=off  Timeout=10  SampleTime=0.01  SimulateUsing=Interpreted execution
  Unused_Receive_Status : Terminator
  Unused_Request_List_Msg : Terminator
  wires:
  UDP_Receive_QGC/2 -> Unused_Receive_Status/1
  Decode_Request_List/2 -> Unused_Request_List_Msg/1
  Decode_Request_Item/2 -> Select_Request_Seq/1
  UDP_Receive_QGC/1 -> Decode_Request_List/1, Decode_Request_Item/1
  Decode_Request_List/1 -> Send_Mission_Count/Enable  "status"
  Select_Request_Seq/1 -> Send_Mission_Item/1(Requested_Sequence)  "<seq>"
  Decode_Request_Item/1 -> Send_Mission_Item/Enable  "status"

== system Kirov_physics/SendState/Mavlink/WGS84 ==
  pos_O_m : Inport
  initial_pos : Inport  Port=2
  Add : Sum
  Data Type Conversion : DataTypeConversion  OutDataTypeStr=double  SaturateOnIntegerOverflow=off  RndMeth=Floor
  Delay : Delay  DelayLength=1
  Delay1 : Delay  DelayLength=1  InitialConditionSource=Input port  InitialCondition=[lat_0;lon_0;hgt_0]
      settings: InputPortMap=u0,p4
  Demux : Demux  Outputs=3
  Divide : Product  Inputs=/*
  Mux : Mux  Inputs=3
  Subtract : Sum  Inputs=+-
  Terminator : Terminator
  WGS84_Derivative : Subsystem
  Zero_Value_Exclusion : Subsystem
  WGS84_Pos : Outport  VectorParamsAs1DForOutWhenUnconnected=off
  wires:
  pos_O_m/1 -> Data Type Conversion/1
  Delay/1 -> Subtract/2
  WGS84_Derivative/1(dx_dlat) -> Mux/1
  Mux/1 -> Zero_Value_Exclusion/1(u)
  Zero_Value_Exclusion/1(y) -> Divide/1
  WGS84_Derivative/3(dz_dh) -> Mux/3
  WGS84_Derivative/2(dy_dlon) -> Mux/2
  Subtract/1 -> Divide/2
  Divide/1 -> Add/1
  Delay1/1 -> Add/2, Demux/1
  Add/1 -> Delay1/1, WGS84_Pos/1
  Demux/1 -> WGS84_Derivative/1(lat_0)
  Demux/3 -> WGS84_Derivative/2(h_0)
  Demux/2 -> Terminator/1
  Data Type Conversion/1 -> Delay/1, Subtract/1
  initial_pos/1 -> Delay1/2
